simulink model "rom"  (R2026b)
settings: Solver=daessc  StopTime=60  FixedStep=0.05
libraries: fl_lib x12, ee_lib x6, nesl_utility x3
settings Model: Creator=Theof  LastModifiedBy=Theof
settings SolverCC: MaxConsecutiveMinStep=20
settings SimscapeCC: SimscapeLogType=all  SimscapeNominalValues="[{\"value\":\"1\",\"unit\":\"A\"},{\"value\":\"1\",\"unit\":\"bar\"},{\"value\":\"1\",\"unit\":\"cm^2\"},{\"value\":\"1\",\"unit\":\"cm^3/s\"},{\"value\":\"1\",\"unit\":\"kJ/kg\"},{\"value\":\"1\",\"unit\":\"kW\"},{\"value\":\"1\",\"unit\":\"l\"},{\"value\":\"1\",\"unit\":\"N\"},{\"value\":\"1\",\"unit\":\"N*m\"},{\"value\":\"1\",\"unit\":\"V\"},{\"value\":\"0.001\",\"unit\":\"Wb\"}]"  SimscapeUseEnergyAccounting=off

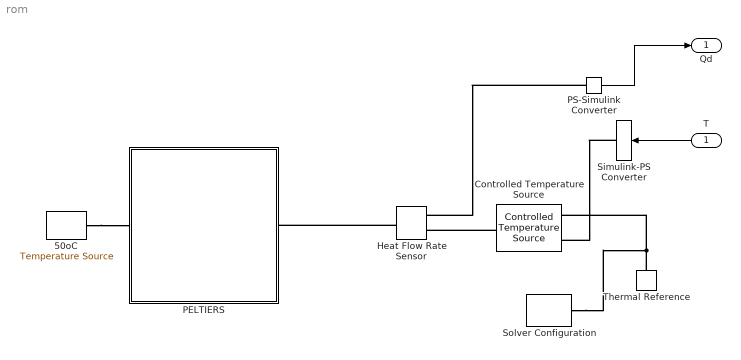
== system rom ==
  T : Inport
  50oC : fl_lib/Thermal/Thermal Sources/Temperature Source  temperature=323 K
  Controlled Temperature Source : fl_lib/Thermal/Thermal Sources/Controlled Temperature Source
  Heat Flow Rate Sensor : fl_lib/Thermal/Thermal Sensors/Heat Flow Rate Sensor
  PELTIERS : Subsystem  mask{vpel=6, rpel=0.1}
      mask prompts: vpel "Voltage"; rpel "Series Resistor"
      mask DialogControl DescGroupVar Prompt: Peltier
  PS-Simulink Converter : nesl_utility/PS-Simulink Converter  PhysicalDomain=network_engine_domain  SubClassName=ps_output  LeftPortType=input  RightPortType=output  PseudoPeriodic=off  Frequencies=[]  VectorFormat=inherit  Unit=inherit  AffineConversion=off
  Simulink-PS Converter : nesl_utility/Simulink-PS Converter  PhysicalDomain=network_engine_domain  SubClassName=ps_input  LeftPortType=input  RightPortType=output  PseudoPeriodic=off  Frequencies=[]  NoiseDistribution=none  NoiseParameters=[]  Unit=1  AffineConversion=off  FilteringAndDerivatives=filter  SimscapeFilterOrder=1  InputFilterTimeConstant=1e-4  UdotUserProvided=0
  Solver Configuration : nesl_utility/Solver Configuration  PhysicalDomain=network_engine_domain  SubClassName=solver  LeftPortType=input  RightPortType=generic  Tones=[]  Harmonics=[]  SimulateNoise=off  Profile=off  UseLocalSampling=off  EnableSwitchedLinearOptims=on  FrequencyDomain=off  UseCCode=off  RelTol=0.001  AbsTol=0.001  MinStep=1e-09  ToWorkspace=off  RevertToSquareIcSolve=off  NumHomotopyIterations=100  PhasorMode=off  PhasorModeNumHarmonics=1  ConsistencySolver=NEWTON_XTOL_AFTER_FTOL  CanonicalOrdering=UNORDERED  OptimizeIntermediates=UNOPTIMIZED  MulticoreSolverChoice=BACKWARD_EULER  IndexReductionMethod=DerivativeReplacement  DoDC=off  ResidualTolerance=1e-09  ConsistencyTolSource=GLOBAL  ConsistencyAbsTol=0.001  ConsistencyRelTol=0.001  ConsistencyTolFactor=0.001  UseLocalSolver=off  LocalSolverChoice=NE_BACKWARD_EULER_ADVANCER  ResolveIndetEquations=on  FunctionEvalNumThread=1  LocalSolverSampleTime=0.5  DoFixedCost=off  MaxNonlinIter=3  MaxModeIter=2  ComputeImpulses=off  ImpulseIterations=2  LinearAlgebra=auto  LinearAlgebraNumThread=0  EquationFormulation=NE_TIME_EF  DelaysMemoryBudget=1024  AutomaticFiltering=on  FilteringTimeConstant=0.001  PartitionStorageMethod=AS_NEEDED  PartitionMemoryBudget=1024  PartitionMethod=BALANCED  MultibodyUseLocalSolver=off  MultibodyLocalSolverChoice=ODE1  MultibodyLocalSolverSampleTime=0.001
  Thermal Reference : fl_lib/Thermal/Thermal Elements/Thermal Reference
  Qd : Outport
  wires:
  T/1 -> Simulink-PS Converter/1
  PS-Simulink Converter/1 -> Qd/1
  connections:
  Simulink-PS Converter/RConn1 -- Controlled Temperature Source/RConn1
  PS-Simulink Converter/LConn1 -- Heat Flow Rate Sensor/RConn1
  Controlled Temperature Source/LConn1 -- Heat Flow Rate Sensor/RConn2
  Thermal Reference/LConn1 -- Solver Configuration/RConn1 -- Controlled Temperature Source/RConn2
  Heat Flow Rate Sensor/LConn1 -- PELTIERS/RConn1
  50oC/LConn1 -- PELTIERS/LConn1

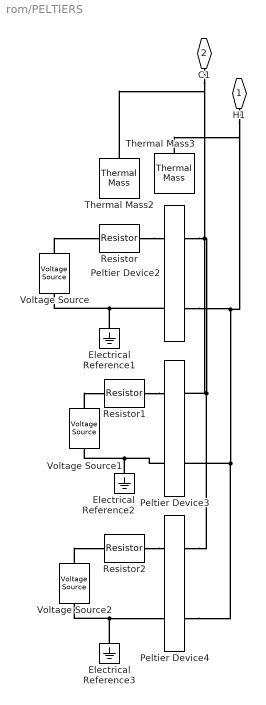
== system rom/PELTIERS ==
  Electrical Reference1 : fl_lib/Electrical/Electrical Elements/Electrical Reference
  Electrical Reference2 : fl_lib/Electrical/Electrical Elements/Electrical Reference
  Electrical Reference3 : fl_lib/Electrical/Electrical Elements/Electrical Reference
  Peltier Device2 : ee_lib/Sensors & Transducers/Peltier Device  alpha=0.053 V/K  R=2 Ohm  K=1/2 W/K
  Peltier Device3 : ee_lib/Sensors & Transducers/Peltier Device  alpha=0.053 V/K  R=2 Ohm  K=1/2 W/K
  Peltier Device4 : ee_lib/Sensors & Transducers/Peltier Device  alpha=0.053 V/K  R=2 Ohm  K=1/2 W/K
  Resistor : fl_lib/Electrical/Electrical Elements/Resistor  R=rpel Ohm  i_specify=off  i_priority=None  i=0 A  i_nominal_specify=off  i_nominal_value=1  i_nominal_unit=A  v_specify=off  v_priority=None  v=0 V  v_nominal_specify=off  v_nominal_value=1  v_nominal_unit=V
  Resistor1 : fl_lib/Electrical/Electrical Elements/Resistor  R=rpel Ohm  i_specify=off  i_priority=None  i=0 A  i_nominal_specify=off  i_nominal_value=1  i_nominal_unit=A  v_specify=off  v_priority=None  v=0 V  v_nominal_specify=off  v_nominal_value=1  v_nominal_unit=V
  Resistor2 : fl_lib/Electrical/Electrical Elements/Resistor  R=rpel Ohm  i_specify=off  i_priority=None  i=0 A  i_nominal_specify=off  i_nominal_value=1  i_nominal_unit=A  v_specify=off  v_priority=None  v=0 V  v_nominal_specify=off  v_nominal_value=1  v_nominal_unit=V
  Thermal Mass2 : fl_lib/Thermal/Thermal Elements/Thermal Mass  mass_type=foundation.enum.constant_variable.constant  mass=(0.025/2)*3 kg  sp_heat=600 J/(K*kg)  mass_min=1e-6 kg  num_ports=foundation.enum.numPorts2.one  m_specify=off  m_priority=High  m=1 kg  m_nominal_specify=off  m_nominal_value=1  m_nominal_unit=kg  T_specify=on  T_priority=High  T=303 K  T_nominal_specify=off  T_nominal_value=1  T_nominal_unit=K  Q_specify=off  Q_priority=None  Q=0 W  Q_nominal_specify=off  Q_nominal_value=1  Q_nominal_unit=W
  Thermal Mass3 : fl_lib/Thermal/Thermal Elements/Thermal Mass  mass_type=foundation.enum.constant_variable.constant  mass=(0.025/2)*3 kg  sp_heat=600 J/(K*kg)  mass_min=1e-6 kg  num_ports=foundation.enum.numPorts2.one  m_specify=off  m_priority=High  m=1 kg  m_nominal_specify=off  m_nominal_value=1  m_nominal_unit=kg  T_specify=on  T_priority=High  T=303 K  T_nominal_specify=off  T_nominal_value=1  T_nominal_unit=K  Q_specify=off  Q_priority=None  Q=0 W  Q_nominal_specify=off  Q_nominal_value=1  Q_nominal_unit=W
  Voltage Source : ee_lib/Sources/Voltage Source  dc_voltage=vpel V  ac_voltage=0 V  ac_shift=0 rad  ac_frequency=60 Hz  noise_mode=ee.enum.sources.noise.Disabled  PSD=0 V^2/Hz  sample_time=1e-3 s  repeatability=ee.enum.sources.repeatability.NotRepeatable  user_seed=0  auto_seed=3499211588  i_specify=off  i_priority=None  i=0 A  i_nominal_specify=off  i_nominal_value=1  i_nominal_unit=A  v_specify=off  v_priority=None  v=0 V  v_nominal_specify=off  v_nominal_value=1  v_nominal_unit=V
  Voltage Source1 : ee_lib/Sources/Voltage Source  dc_voltage=vpel V  ac_voltage=0 V  ac_shift=0 rad  ac_frequency=60 Hz  noise_mode=ee.enum.sources.noise.Disabled  PSD=0 V^2/Hz  sample_time=1e-3 s  repeatability=ee.enum.sources.repeatability.NotRepeatable  user_seed=0  auto_seed=3890346746  i_specify=off  i_priority=None  i=0 A  i_nominal_specify=off  i_nominal_value=1  i_nominal_unit=A  v_specify=off  v_priority=None  v=0 V  v_nominal_specify=off  v_nominal_value=1  v_nominal_unit=V
  Voltage Source2 : ee_lib/Sources/Voltage Source  dc_voltage=vpel V  ac_voltage=0 V  ac_shift=0 rad  ac_frequency=60 Hz  noise_mode=ee.enum.sources.noise.Disabled  PSD=0 V^2/Hz  sample_time=1e-3 s  repeatability=ee.enum.sources.repeatability.NotRepeatable  user_seed=0  auto_seed=545404223  i_specify=off  i_priority=None  i=0 A  i_nominal_specify=off  i_nominal_value=1  i_nominal_unit=A  v_specify=off  v_priority=None  v=0 V  v_nominal_specify=off  v_nominal_value=1  v_nominal_unit=V
  H1 : PMIOPort  Side=Left
  C1 : PMIOPort  Port=2  Side=Right
  connections:
  Peltier Device4/RConn1 -- Thermal Mass2/LConn1 -- C1/RConn1 -- Peltier Device2/RConn1 -- Peltier Device3/RConn1
  Peltier Device4/RConn2 -- Thermal Mass3/LConn1 -- H1/RConn1 -- Peltier Device2/RConn2 -- Peltier Device3/RConn2
  Electrical Reference1/LConn1 -- Peltier Device2/LConn2 -- Voltage Source/RConn1
  Electrical Reference2/LConn1 -- Peltier Device3/LConn2 -- Voltage Source1/RConn1
  Electrical Reference3/LConn1 -- Peltier Device4/LConn2 -- Voltage Source2/RConn1
  Resistor/RConn1 -- Peltier Device2/LConn1
  Voltage Source/LConn1 -- Resistor/LConn1
  Resistor1/RConn1 -- Peltier Device3/LConn1
  Voltage Source1/LConn1 -- Resistor1/LConn1
  Resistor2/RConn1 -- Peltier Device4/LConn1
  Voltage Source2/LConn1 -- Resistor2/LConn1
